simulink model "MMC_phase_hackathon_circuit4_HAAS_20260216"  (R2024b)
settings: Solver=FixedStepDiscrete  StartTime=t_init_sim  StopTime=sim_time  FixedStep=Ts  RelTol=1e-3
values from neighbouring files (symbols this model uses):
  a = 1    [param_phase_circuit4_20260216.m]
  C1low1_active = 1    [script_MMC_phase_circuit4_twist_20260216.m]
  C2low1_active = 1    [script_MMC_phase_circuit4_twist_20260216.m]
  C_bus = 4400e-6    (= 0.0044)    [param_phase_circuit4_20260216.m]
  C_M_extra = C_m-twist_high_side_C    [param_phase_circuit4_20260216.m]
  duty_cycle = 0.95    [script_MMC_phase_circuit4_twist_20260216.m]
  f0 = 50    [param_phase_circuit4_20260216.m]
  feeder_current_lower_rate_limit = -10    [script_MMC_phase_circuit4_twist_20260216.m]    (also in twist_parameters.m = -500)
  feeder_current_tab = [0.328 0.217 0.162 0.132 0.109 0.094 0.083 0.075 0.068 0.062 0.058 0.054 ... (42 elements, 14x3)]    [feeder_current.mat]
  feeder_current_upper_rate_limit = 0.386/(20e-3)    (= 19.3)    [twist_parameters.m]
  is6VExternallySupplied = true    [script_MMC_phase_circuit4_twist_20260216.m]
  isFeederJumperOpen = true    [script_MMC_phase_circuit4_twist_20260216.m]
  L_arm = 30e-3    (= 0.03)    [param_phase_circuit4_20260216.m]
  m = 1    [param_phase_circuit4_20260216.m]
  N = 5    [param_phase_circuit4_20260216.m]
  power_losses = false    [script_MMC_phase_circuit4_twist_20260216.m]
  R = 30    [param_phase_circuit4_20260216.m]
  source_V = 0    [script_MMC_phase_circuit4_twist_20260216.m]
  time_charge = 0.1    [script_MMC_phase_circuit4_twist_20260216.m]
  time_decharge = 1.5    [script_MMC_phase_circuit4_twist_20260216.m]
  Ts = 5e-7    (= 5e-07)    [script_MMC_phase_circuit4_twist_20260216.m]
  twist_data_acquisition_delay = 50e-9    (= 5e-08)    [script_MMC_phase_circuit4_twist_20260216.m]    (also in twist_parameters.m)
  twist_data_sampling_period = 1/twist_freq_data_sampling    (= 5e-05)    [script_MMC_phase_circuit4_twist_20260216.m]    (also in twist_parameters.m)
  twist_dead_time = 200e-9    (= 2e-07)    [twist_parameters.m]
  twist_freq_switching = 200e3    (= 200000)    [twist_parameters.m]
  twist_high_side_adc_R = 1/(1/2e6 + 1/2e6 + 1/(330e3+5.6e3))    (= 251272.836178)    [twist_parameters.m]
  twist_high_side_C = 33e-6*4 + 4.7e-6*12    (= 0.0001884)    [twist_parameters.m]
  twist_high_side_feeder_R = 47e3+4.7e3    (= 51700)    [twist_parameters.m]
  twist_high_side_rC = 0.1    [twist_parameters.m]
  twist_low_side_adc_R = 150e3+470    (= 150470)    [twist_parameters.m]
  twist_low_side_C_ceramic = 3*4.7e-6    (= 1.41e-05)    [twist_parameters.m]
  twist_low_side_C_electrolytic = 47e-6    (= 4.7e-05)    [twist_parameters.m]
  twist_low_side_L = 33e-6    (= 3.3e-05)    [twist_parameters.m]
  twist_low_side_rC = 700e-3    (= 0.7)    [twist_parameters.m]
  twist_low_side_rL = 20e-3    (= 0.02)    [twist_parameters.m]
  twist_R_VCC = (tau_VCC/twist_high_side_C  - twist_high_side_rC)/(1-(tau_VCC/twist_high_side_C - twist_high_side_rC)/R_parallel)    (= 1110.74997822)    [twist_parameters.m]
  VDC = 48    [param_phase_circuit4_20260216.m]
undefined symbols (not defined in the file or in its folder): C_SM, feeder_current, gcbh, sps_rtmsupport, twist_low_side_lC
libraries: spsSeriesRLCBranchLib x135, spsTriangleGeneratorLib x60, spsMosfetLib x60, spsVoltageMeasurementLib x55, spsCurrentMeasurementLib x43, spsControlledCurrentSourceLib x30, spsDiodeLib x22, spsIdealSwitchLib x20, spsControlledVoltageSourceLib x1, spsGroundLib x1, spsMeanLib x1, spspowerguiLib x1
(part 11 of 18)

== system MMC_phase_hackathon_circuit4_HAAS_20260216/ /HB Twist M10/Twist Power Block/HRTimA_1/PWM Generator (2-Level)/Modulator type ==
  Cr : Inport
  Uref : Inport  Port=2
  Full Bridge Bipolar : Subsystem  VariantControl=FullBridgeBipolar
  Full Bridge Unipolar : Subsystem  VariantControl=FullBridgeUnipolar
  One Three Phase Bridge : Subsystem  VariantControl=OneThreePhaseBridge
  P : Outport  VectorParamsAs1DForOutWhenUnconnected=off

== system MMC_phase_hackathon_circuit4_HAAS_20260216/ /HB Twist M10/Twist Power Block/HRTimA_1/PWM Generator (2-Level)/Reference signal ==
  Uref : Inport
  External : Subsystem  VariantControl=External
  Internal : Subsystem  VariantControl=Internal
  Uref_In : Outport  VectorParamsAs1DForOutWhenUnconnected=off

== system MMC_phase_hackathon_circuit4_HAAS_20260216/ /HB Twist M10/Twist Power Block/HRTimA_1/PWM Generator (2-Level)/Sampling ==
  wt : Inport
  Uref : Inport  Port=2
  Sync Asymmetrical : Subsystem  VariantControl=SyncAsymmetrical
  Sync Natural : Subsystem  VariantControl=SyncNatural
  Sync Symmetrical : Subsystem  VariantControl=SyncSymmetrical
  Unsync Asymmetrical : Subsystem  VariantControl=UnsyncAsymmetrical
  Unsync Natural : Subsystem  VariantControl=UnsyncNatural
  Unsync Symmetrical : Subsystem  VariantControl=UnsyncSymmetrical
  Cr : Outport  VectorParamsAs1DForOutWhenUnconnected=off
  Uref* : Outport  Port=2  VectorParamsAs1DForOutWhenUnconnected=off

== system MMC_phase_hackathon_circuit4_HAAS_20260216/ /HB Twist M10/Twist Power Block/HRTimA_2/PWM Generator (2-Level)/Cr_MinMax ==
  MinMax : Inport
  Cr : Inport  Port=2
  Add3 : Sum  Inputs=-+
  Add4 : Sum  Inputs=+++
  Demux : Demux  Outputs=2
  Gain1 : Gain  Gain=0.5
  MUL1 : Product  Inputs=**
  Cr* : Outport  VectorParamsAs1DForOutWhenUnconnected=off
  wires:
  Add3/1 -> Gain1/1
  MinMax/1 -> Demux/1
  Demux/1 -> Add4/1, Add3/1
  Demux/2 -> Add3/2
  Gain1/1 -> Add4/3, MUL1/2
  Cr/1 -> MUL1/1
  Add4/1 -> Cr*/1
  MUL1/1 -> Add4/2

== system MMC_phase_hackathon_circuit4_HAAS_20260216/ /HB Twist M10/Twist Power Block/HRTimA_2/PWM Generator (2-Level)/Modulator type ==
  Cr : Inport
  Uref : Inport  Port=2
  Full Bridge Bipolar : Subsystem  VariantControl=FullBridgeBipolar
  Full Bridge Unipolar : Subsystem  VariantControl=FullBridgeUnipolar
  One Three Phase Bridge : Subsystem  VariantControl=OneThreePhaseBridge
  P : Outport  VectorParamsAs1DForOutWhenUnconnected=off

== system MMC_phase_hackathon_circuit4_HAAS_20260216/ /HB Twist M10/Twist Power Block/HRTimA_2/PWM Generator (2-Level)/Reference signal ==
  Uref : Inport
  External : Subsystem  VariantControl=External
  Internal : Subsystem  VariantControl=Internal
  Uref_In : Outport  VectorParamsAs1DForOutWhenUnconnected=off

== system MMC_phase_hackathon_circuit4_HAAS_20260216/ /HB Twist M10/Twist Power Block/HRTimA_2/PWM Generator (2-Level)/Sampling ==
  wt : Inport
  Uref : Inport  Port=2
  Sync Asymmetrical : Subsystem  VariantControl=SyncAsymmetrical
  Sync Natural : Subsystem  VariantControl=SyncNatural
  Sync Symmetrical : Subsystem  VariantControl=SyncSymmetrical
  Unsync Asymmetrical : Subsystem  VariantControl=UnsyncAsymmetrical
  Unsync Natural : Subsystem  VariantControl=UnsyncNatural
  Unsync Symmetrical : Subsystem  VariantControl=UnsyncSymmetrical
  Cr : Outport  VectorParamsAs1DForOutWhenUnconnected=off
  Uref* : Outport  Port=2  VectorParamsAs1DForOutWhenUnconnected=off

== system MMC_phase_hackathon_circuit4_HAAS_20260216/ /HB Twist M2/Twist Power Block/HRTimA_1/PWM Generator (2-Level)/Cr_MinMax ==
  MinMax : Inport
  Cr : Inport  Port=2
  Add3 : Sum  Inputs=-+
  Add4 : Sum  Inputs=+++
  Demux : Demux  Outputs=2
  Gain1 : Gain  Gain=0.5
  MUL1 : Product  Inputs=**
  Cr* : Outport  VectorParamsAs1DForOutWhenUnconnected=off
  wires:
  Add3/1 -> Gain1/1
  MinMax/1 -> Demux/1
  Demux/1 -> Add4/1, Add3/1
  Demux/2 -> Add3/2
  Gain1/1 -> Add4/3, MUL1/2
  Cr/1 -> MUL1/1
  Add4/1 -> Cr*/1
  MUL1/1 -> Add4/2

== system MMC_phase_hackathon_circuit4_HAAS_20260216/ /HB Twist M2/Twist Power Block/HRTimA_1/PWM Generator (2-Level)/Modulator type ==
  Cr : Inport
  Uref : Inport  Port=2
  Full Bridge Bipolar : Subsystem  VariantControl=FullBridgeBipolar
  Full Bridge Unipolar : Subsystem  VariantControl=FullBridgeUnipolar
  One Three Phase Bridge : Subsystem  VariantControl=OneThreePhaseBridge
  P : Outport  VectorParamsAs1DForOutWhenUnconnected=off

== system MMC_phase_hackathon_circuit4_HAAS_20260216/ /HB Twist M2/Twist Power Block/HRTimA_1/PWM Generator (2-Level)/Reference signal ==
  Uref : Inport
  External : Subsystem  VariantControl=External
  Internal : Subsystem  VariantControl=Internal
  Uref_In : Outport  VectorParamsAs1DForOutWhenUnconnected=off

== system MMC_phase_hackathon_circuit4_HAAS_20260216/ /HB Twist M2/Twist Power Block/HRTimA_1/PWM Generator (2-Level)/Sampling ==
  wt : Inport
  Uref : Inport  Port=2
  Sync Asymmetrical : Subsystem  VariantControl=SyncAsymmetrical
  Sync Natural : Subsystem  VariantControl=SyncNatural
  Sync Symmetrical : Subsystem  VariantControl=SyncSymmetrical
  Unsync Asymmetrical : Subsystem  VariantControl=UnsyncAsymmetrical
  Unsync Natural : Subsystem  VariantControl=UnsyncNatural
  Unsync Symmetrical : Subsystem  VariantControl=UnsyncSymmetrical
  Cr : Outport  VectorParamsAs1DForOutWhenUnconnected=off
  Uref* : Outport  Port=2  VectorParamsAs1DForOutWhenUnconnected=off

== system MMC_phase_hackathon_circuit4_HAAS_20260216/ /HB Twist M2/Twist Power Block/HRTimA_2/PWM Generator (2-Level)/Cr_MinMax ==
  MinMax : Inport
  Cr : Inport  Port=2
  Add3 : Sum  Inputs=-+
  Add4 : Sum  Inputs=+++
  Demux : Demux  Outputs=2
  Gain1 : Gain  Gain=0.5
  MUL1 : Product  Inputs=**
  Cr* : Outport  VectorParamsAs1DForOutWhenUnconnected=off
  wires:
  Add3/1 -> Gain1/1
  MinMax/1 -> Demux/1
  Demux/1 -> Add4/1, Add3/1
  Demux/2 -> Add3/2
  Gain1/1 -> Add4/3, MUL1/2
  Cr/1 -> MUL1/1
  Add4/1 -> Cr*/1
  MUL1/1 -> Add4/2

== system MMC_phase_hackathon_circuit4_HAAS_20260216/ /HB Twist M2/Twist Power Block/HRTimA_2/PWM Generator (2-Level)/Modulator type ==
  Cr : Inport
  Uref : Inport  Port=2
  Full Bridge Bipolar : Subsystem  VariantControl=FullBridgeBipolar
  Full Bridge Unipolar : Subsystem  VariantControl=FullBridgeUnipolar
  One Three Phase Bridge : Subsystem  VariantControl=OneThreePhaseBridge
  P : Outport  VectorParamsAs1DForOutWhenUnconnected=off

== system MMC_phase_hackathon_circuit4_HAAS_20260216/ /HB Twist M2/Twist Power Block/HRTimA_2/PWM Generator (2-Level)/Reference signal ==
  Uref : Inport
  External : Subsystem  VariantControl=External
  Internal : Subsystem  VariantControl=Internal
  Uref_In : Outport  VectorParamsAs1DForOutWhenUnconnected=off

== system MMC_phase_hackathon_circuit4_HAAS_20260216/ /HB Twist M2/Twist Power Block/HRTimA_2/PWM Generator (2-Level)/Sampling ==
  wt : Inport
  Uref : Inport  Port=2
  Sync Asymmetrical : Subsystem  VariantControl=SyncAsymmetrical
  Sync Natural : Subsystem  VariantControl=SyncNatural
  Sync Symmetrical : Subsystem  VariantControl=SyncSymmetrical
  Unsync Asymmetrical : Subsystem  VariantControl=UnsyncAsymmetrical
  Unsync Natural : Subsystem  VariantControl=UnsyncNatural
  Unsync Symmetrical : Subsystem  VariantControl=UnsyncSymmetrical
  Cr : Outport  VectorParamsAs1DForOutWhenUnconnected=off
  Uref* : Outport  Port=2  VectorParamsAs1DForOutWhenUnconnected=off

== system MMC_phase_hackathon_circuit4_HAAS_20260216/ /HB Twist M3/Twist Power Block/HRTimA_1/PWM Generator (2-Level)/Cr_MinMax ==
  MinMax : Inport
  Cr : Inport  Port=2
  Add3 : Sum  Inputs=-+
  Add4 : Sum  Inputs=+++
  Demux : Demux  Outputs=2
  Gain1 : Gain  Gain=0.5
  MUL1 : Product  Inputs=**
  Cr* : Outport  VectorParamsAs1DForOutWhenUnconnected=off
  wires:
  Add3/1 -> Gain1/1
  MinMax/1 -> Demux/1
  Demux/1 -> Add4/1, Add3/1
  Demux/2 -> Add3/2
  Gain1/1 -> Add4/3, MUL1/2
  Cr/1 -> MUL1/1
  Add4/1 -> Cr*/1
  MUL1/1 -> Add4/2

== system MMC_phase_hackathon_circuit4_HAAS_20260216/ /HB Twist M3/Twist Power Block/HRTimA_1/PWM Generator (2-Level)/Modulator type ==
  Cr : Inport
  Uref : Inport  Port=2
  Full Bridge Bipolar : Subsystem  VariantControl=FullBridgeBipolar
  Full Bridge Unipolar : Subsystem  VariantControl=FullBridgeUnipolar
  One Three Phase Bridge : Subsystem  VariantControl=OneThreePhaseBridge
  P : Outport  VectorParamsAs1DForOutWhenUnconnected=off

== system MMC_phase_hackathon_circuit4_HAAS_20260216/ /HB Twist M3/Twist Power Block/HRTimA_1/PWM Generator (2-Level)/Reference signal ==
  Uref : Inport
  External : Subsystem  VariantControl=External
  Internal : Subsystem  VariantControl=Internal
  Uref_In : Outport  VectorParamsAs1DForOutWhenUnconnected=off

== system MMC_phase_hackathon_circuit4_HAAS_20260216/ /HB Twist M3/Twist Power Block/HRTimA_1/PWM Generator (2-Level)/Sampling ==
  wt : Inport
  Uref : Inport  Port=2
  Sync Asymmetrical : Subsystem  VariantControl=SyncAsymmetrical
  Sync Natural : Subsystem  VariantControl=SyncNatural
  Sync Symmetrical : Subsystem  VariantControl=SyncSymmetrical
  Unsync Asymmetrical : Subsystem  VariantControl=UnsyncAsymmetrical
  Unsync Natural : Subsystem  VariantControl=UnsyncNatural
  Unsync Symmetrical : Subsystem  VariantControl=UnsyncSymmetrical
  Cr : Outport  VectorParamsAs1DForOutWhenUnconnected=off
  Uref* : Outport  Port=2  VectorParamsAs1DForOutWhenUnconnected=off

== system MMC_phase_hackathon_circuit4_HAAS_20260216/ /HB Twist M3/Twist Power Block/HRTimA_2/PWM Generator (2-Level)/Cr_MinMax ==
  MinMax : Inport
  Cr : Inport  Port=2
  Add3 : Sum  Inputs=-+
  Add4 : Sum  Inputs=+++
  Demux : Demux  Outputs=2
  Gain1 : Gain  Gain=0.5
  MUL1 : Product  Inputs=**
  Cr* : Outport  VectorParamsAs1DForOutWhenUnconnected=off
  wires:
  Add3/1 -> Gain1/1
  MinMax/1 -> Demux/1
  Demux/1 -> Add4/1, Add3/1
  Demux/2 -> Add3/2
  Gain1/1 -> Add4/3, MUL1/2
  Cr/1 -> MUL1/1
  Add4/1 -> Cr*/1
  MUL1/1 -> Add4/2

== system MMC_phase_hackathon_circuit4_HAAS_20260216/ /HB Twist M3/Twist Power Block/HRTimA_2/PWM Generator (2-Level)/Modulator type ==
  Cr : Inport
  Uref : Inport  Port=2
  Full Bridge Bipolar : Subsystem  VariantControl=FullBridgeBipolar
  Full Bridge Unipolar : Subsystem  VariantControl=FullBridgeUnipolar
  One Three Phase Bridge : Subsystem  VariantControl=OneThreePhaseBridge
  P : Outport  VectorParamsAs1DForOutWhenUnconnected=off

== system MMC_phase_hackathon_circuit4_HAAS_20260216/ /HB Twist M3/Twist Power Block/HRTimA_2/PWM Generator (2-Level)/Reference signal ==
  Uref : Inport
  External : Subsystem  VariantControl=External
  Internal : Subsystem  VariantControl=Internal
  Uref_In : Outport  VectorParamsAs1DForOutWhenUnconnected=off

== system MMC_phase_hackathon_circuit4_HAAS_20260216/ /HB Twist M3/Twist Power Block/HRTimA_2/PWM Generator (2-Level)/Sampling ==
  wt : Inport
  Uref : Inport  Port=2
  Sync Asymmetrical : Subsystem  VariantControl=SyncAsymmetrical
  Sync Natural : Subsystem  VariantControl=SyncNatural
  Sync Symmetrical : Subsystem  VariantControl=SyncSymmetrical
  Unsync Asymmetrical : Subsystem  VariantControl=UnsyncAsymmetrical
  Unsync Natural : Subsystem  VariantControl=UnsyncNatural
  Unsync Symmetrical : Subsystem  VariantControl=UnsyncSymmetrical
  Cr : Outport  VectorParamsAs1DForOutWhenUnconnected=off
  Uref* : Outport  Port=2  VectorParamsAs1DForOutWhenUnconnected=off

== system MMC_phase_hackathon_circuit4_HAAS_20260216/ /HB Twist M4/Twist Power Block/HRTimA_1/PWM Generator (2-Level)/Cr_MinMax ==
  MinMax : Inport
  Cr : Inport  Port=2
  Add3 : Sum  Inputs=-+
  Add4 : Sum  Inputs=+++
  Demux : Demux  Outputs=2
  Gain1 : Gain  Gain=0.5
  MUL1 : Product  Inputs=**
  Cr* : Outport  VectorParamsAs1DForOutWhenUnconnected=off
  wires:
  Add3/1 -> Gain1/1
  MinMax/1 -> Demux/1
  Demux/1 -> Add4/1, Add3/1
  Demux/2 -> Add3/2
  Gain1/1 -> Add4/3, MUL1/2
  Cr/1 -> MUL1/1
  Add4/1 -> Cr*/1
  MUL1/1 -> Add4/2

== system MMC_phase_hackathon_circuit4_HAAS_20260216/ /HB Twist M4/Twist Power Block/HRTimA_1/PWM Generator (2-Level)/Modulator type ==
  Cr : Inport
  Uref : Inport  Port=2
  Full Bridge Bipolar : Subsystem  VariantControl=FullBridgeBipolar
  Full Bridge Unipolar : Subsystem  VariantControl=FullBridgeUnipolar
  One Three Phase Bridge : Subsystem  VariantControl=OneThreePhaseBridge
  P : Outport  VectorParamsAs1DForOutWhenUnconnected=off

== system MMC_phase_hackathon_circuit4_HAAS_20260216/ /HB Twist M4/Twist Power Block/HRTimA_1/PWM Generator (2-Level)/Reference signal ==
  Uref : Inport
  External : Subsystem  VariantControl=External
  Internal : Subsystem  VariantControl=Internal
  Uref_In : Outport  VectorParamsAs1DForOutWhenUnconnected=off

== system MMC_phase_hackathon_circuit4_HAAS_20260216/ /HB Twist M4/Twist Power Block/HRTimA_1/PWM Generator (2-Level)/Sampling ==
  wt : Inport
  Uref : Inport  Port=2
  Sync Asymmetrical : Subsystem  VariantControl=SyncAsymmetrical
  Sync Natural : Subsystem  VariantControl=SyncNatural
  Sync Symmetrical : Subsystem  VariantControl=SyncSymmetrical
  Unsync Asymmetrical : Subsystem  VariantControl=UnsyncAsymmetrical
  Unsync Natural : Subsystem  VariantControl=UnsyncNatural
  Unsync Symmetrical : Subsystem  VariantControl=UnsyncSymmetrical
  Cr : Outport  VectorParamsAs1DForOutWhenUnconnected=off
  Uref* : Outport  Port=2  VectorParamsAs1DForOutWhenUnconnected=off

== system MMC_phase_hackathon_circuit4_HAAS_20260216/ /HB Twist M4/Twist Power Block/HRTimA_2/PWM Generator (2-Level)/Cr_MinMax ==
  MinMax : Inport
  Cr : Inport  Port=2
  Add3 : Sum  Inputs=-+
  Add4 : Sum  Inputs=+++
  Demux : Demux  Outputs=2
  Gain1 : Gain  Gain=0.5
  MUL1 : Product  Inputs=**
  Cr* : Outport  VectorParamsAs1DForOutWhenUnconnected=off
  wires:
  Add3/1 -> Gain1/1
  MinMax/1 -> Demux/1
  Demux/1 -> Add4/1, Add3/1
  Demux/2 -> Add3/2
  Gain1/1 -> Add4/3, MUL1/2
  Cr/1 -> MUL1/1
  Add4/1 -> Cr*/1
  MUL1/1 -> Add4/2

== system MMC_phase_hackathon_circuit4_HAAS_20260216/ /HB Twist M4/Twist Power Block/HRTimA_2/PWM Generator (2-Level)/Modulator type ==
  Cr : Inport
  Uref : Inport  Port=2
  Full Bridge Bipolar : Subsystem  VariantControl=FullBridgeBipolar
  Full Bridge Unipolar : Subsystem  VariantControl=FullBridgeUnipolar
  One Three Phase Bridge : Subsystem  VariantControl=OneThreePhaseBridge
  P : Outport  VectorParamsAs1DForOutWhenUnconnected=off

== system MMC_phase_hackathon_circuit4_HAAS_20260216/ /HB Twist M4/Twist Power Block/HRTimA_2/PWM Generator (2-Level)/Reference signal ==
  Uref : Inport
  External : Subsystem  VariantControl=External
  Internal : Subsystem  VariantControl=Internal
  Uref_In : Outport  VectorParamsAs1DForOutWhenUnconnected=off

== system MMC_phase_hackathon_circuit4_HAAS_20260216/ /HB Twist M4/Twist Power Block/HRTimA_2/PWM Generator (2-Level)/Sampling ==
  wt : Inport
  Uref : Inport  Port=2
  Sync Asymmetrical : Subsystem  VariantControl=SyncAsymmetrical
  Sync Natural : Subsystem  VariantControl=SyncNatural
  Sync Symmetrical : Subsystem  VariantControl=SyncSymmetrical
  Unsync Asymmetrical : Subsystem  VariantControl=UnsyncAsymmetrical
  Unsync Natural : Subsystem  VariantControl=UnsyncNatural
  Unsync Symmetrical : Subsystem  VariantControl=UnsyncSymmetrical
  Cr : Outport  VectorParamsAs1DForOutWhenUnconnected=off
  Uref* : Outport  Port=2  VectorParamsAs1DForOutWhenUnconnected=off

== system MMC_phase_hackathon_circuit4_HAAS_20260216/ /HB Twist M5/Twist Power Block/HRTimA_1/PWM Generator (2-Level)/Cr_MinMax ==
  MinMax : Inport
  Cr : Inport  Port=2
  Add3 : Sum  Inputs=-+
  Add4 : Sum  Inputs=+++
  Demux : Demux  Outputs=2
  Gain1 : Gain  Gain=0.5
  MUL1 : Product  Inputs=**
  Cr* : Outport  VectorParamsAs1DForOutWhenUnconnected=off
  wires:
  Add3/1 -> Gain1/1
  MinMax/1 -> Demux/1
  Demux/1 -> Add4/1, Add3/1
  Demux/2 -> Add3/2
  Gain1/1 -> Add4/3, MUL1/2
  Cr/1 -> MUL1/1
  Add4/1 -> Cr*/1
  MUL1/1 -> Add4/2

== system MMC_phase_hackathon_circuit4_HAAS_20260216/ /HB Twist M5/Twist Power Block/HRTimA_1/PWM Generator (2-Level)/Modulator type ==
  Cr : Inport
  Uref : Inport  Port=2
  Full Bridge Bipolar : Subsystem  VariantControl=FullBridgeBipolar
  Full Bridge Unipolar : Subsystem  VariantControl=FullBridgeUnipolar
  One Three Phase Bridge : Subsystem  VariantControl=OneThreePhaseBridge
  P : Outport  VectorParamsAs1DForOutWhenUnconnected=off

== system MMC_phase_hackathon_circuit4_HAAS_20260216/ /HB Twist M5/Twist Power Block/HRTimA_1/PWM Generator (2-Level)/Reference signal ==
  Uref : Inport
  External : Subsystem  VariantControl=External
  Internal : Subsystem  VariantControl=Internal
  Uref_In : Outport  VectorParamsAs1DForOutWhenUnconnected=off

== system MMC_phase_hackathon_circuit4_HAAS_20260216/ /HB Twist M5/Twist Power Block/HRTimA_1/PWM Generator (2-Level)/Sampling ==
  wt : Inport
  Uref : Inport  Port=2
  Sync Asymmetrical : Subsystem  VariantControl=SyncAsymmetrical
  Sync Natural : Subsystem  VariantControl=SyncNatural
  Sync Symmetrical : Subsystem  VariantControl=SyncSymmetrical
  Unsync Asymmetrical : Subsystem  VariantControl=UnsyncAsymmetrical
  Unsync Natural : Subsystem  VariantControl=UnsyncNatural
  Unsync Symmetrical : Subsystem  VariantControl=UnsyncSymmetrical
  Cr : Outport  VectorParamsAs1DForOutWhenUnconnected=off
  Uref* : Outport  Port=2  VectorParamsAs1DForOutWhenUnconnected=off

== system MMC_phase_hackathon_circuit4_HAAS_20260216/ /HB Twist M5/Twist Power Block/HRTimA_2/PWM Generator (2-Level)/Cr_MinMax ==
  MinMax : Inport
  Cr : Inport  Port=2
  Add3 : Sum  Inputs=-+
  Add4 : Sum  Inputs=+++
  Demux : Demux  Outputs=2
  Gain1 : Gain  Gain=0.5
  MUL1 : Product  Inputs=**
  Cr* : Outport  VectorParamsAs1DForOutWhenUnconnected=off
  wires:
  Add3/1 -> Gain1/1
  MinMax/1 -> Demux/1
  Demux/1 -> Add4/1, Add3/1
  Demux/2 -> Add3/2
  Gain1/1 -> Add4/3, MUL1/2
  Cr/1 -> MUL1/1
  Add4/1 -> Cr*/1
  MUL1/1 -> Add4/2

== system MMC_phase_hackathon_circuit4_HAAS_20260216/ /HB Twist M5/Twist Power Block/HRTimA_2/PWM Generator (2-Level)/Modulator type ==
  Cr : Inport
  Uref : Inport  Port=2
  Full Bridge Bipolar : Subsystem  VariantControl=FullBridgeBipolar
  Full Bridge Unipolar : Subsystem  VariantControl=FullBridgeUnipolar
  One Three Phase Bridge : Subsystem  VariantControl=OneThreePhaseBridge
  P : Outport  VectorParamsAs1DForOutWhenUnconnected=off

== system MMC_phase_hackathon_circuit4_HAAS_20260216/ /HB Twist M5/Twist Power Block/HRTimA_2/PWM Generator (2-Level)/Reference signal ==
  Uref : Inport
  External : Subsystem  VariantControl=External
  Internal : Subsystem  VariantControl=Internal
  Uref_In : Outport  VectorParamsAs1DForOutWhenUnconnected=off

== system MMC_phase_hackathon_circuit4_HAAS_20260216/ /HB Twist M5/Twist Power Block/HRTimA_2/PWM Generator (2-Level)/Sampling ==
  wt : Inport
  Uref : Inport  Port=2
  Sync Asymmetrical : Subsystem  VariantControl=SyncAsymmetrical
  Sync Natural : Subsystem  VariantControl=SyncNatural
  Sync Symmetrical : Subsystem  VariantControl=SyncSymmetrical
  Unsync Asymmetrical : Subsystem  VariantControl=UnsyncAsymmetrical
  Unsync Natural : Subsystem  VariantControl=UnsyncNatural
  Unsync Symmetrical : Subsystem  VariantControl=UnsyncSymmetrical
  Cr : Outport  VectorParamsAs1DForOutWhenUnconnected=off
  Uref* : Outport  Port=2  VectorParamsAs1DForOutWhenUnconnected=off

== system MMC_phase_hackathon_circuit4_HAAS_20260216/ /HB Twist M6/Twist Power Block/HRTimA_1/PWM Generator (2-Level)/Cr_MinMax ==
  MinMax : Inport
  Cr : Inport  Port=2
  Add3 : Sum  Inputs=-+
  Add4 : Sum  Inputs=+++
  Demux : Demux  Outputs=2
  Gain1 : Gain  Gain=0.5
  MUL1 : Product  Inputs=**
  Cr* : Outport  VectorParamsAs1DForOutWhenUnconnected=off
  wires:
  Add3/1 -> Gain1/1
  MinMax/1 -> Demux/1
  Demux/1 -> Add4/1, Add3/1
  Demux/2 -> Add3/2
  Gain1/1 -> Add4/3, MUL1/2
  Cr/1 -> MUL1/1
  Add4/1 -> Cr*/1
  MUL1/1 -> Add4/2

== system MMC_phase_hackathon_circuit4_HAAS_20260216/ /HB Twist M6/Twist Power Block/HRTimA_1/PWM Generator (2-Level)/Modulator type ==
  Cr : Inport
  Uref : Inport  Port=2
  Full Bridge Bipolar : Subsystem  VariantControl=FullBridgeBipolar
  Full Bridge Unipolar : Subsystem  VariantControl=FullBridgeUnipolar
  One Three Phase Bridge : Subsystem  VariantControl=OneThreePhaseBridge
  P : Outport  VectorParamsAs1DForOutWhenUnconnected=off

== system MMC_phase_hackathon_circuit4_HAAS_20260216/ /HB Twist M6/Twist Power Block/HRTimA_1/PWM Generator (2-Level)/Reference signal ==
  Uref : Inport
  External : Subsystem  VariantControl=External
  Internal : Subsystem  VariantControl=Internal
  Uref_In : Outport  VectorParamsAs1DForOutWhenUnconnected=off

== system MMC_phase_hackathon_circuit4_HAAS_20260216/ /HB Twist M6/Twist Power Block/HRTimA_1/PWM Generator (2-Level)/Sampling ==
  wt : Inport
  Uref : Inport  Port=2
  Sync Asymmetrical : Subsystem  VariantControl=SyncAsymmetrical
  Sync Natural : Subsystem  VariantControl=SyncNatural
  Sync Symmetrical : Subsystem  VariantControl=SyncSymmetrical
  Unsync Asymmetrical : Subsystem  VariantControl=UnsyncAsymmetrical
  Unsync Natural : Subsystem  VariantControl=UnsyncNatural
  Unsync Symmetrical : Subsystem  VariantControl=UnsyncSymmetrical
  Cr : Outport  VectorParamsAs1DForOutWhenUnconnected=off
  Uref* : Outport  Port=2  VectorParamsAs1DForOutWhenUnconnected=off

== system MMC_phase_hackathon_circuit4_HAAS_20260216/ /HB Twist M6/Twist Power Block/HRTimA_2/PWM Generator (2-Level)/Cr_MinMax ==
  MinMax : Inport
  Cr : Inport  Port=2
  Add3 : Sum  Inputs=-+
  Add4 : Sum  Inputs=+++
  Demux : Demux  Outputs=2
  Gain1 : Gain  Gain=0.5
  MUL1 : Product  Inputs=**
  Cr* : Outport  VectorParamsAs1DForOutWhenUnconnected=off
  wires:
  Add3/1 -> Gain1/1
  MinMax/1 -> Demux/1
  Demux/1 -> Add4/1, Add3/1
  Demux/2 -> Add3/2
  Gain1/1 -> Add4/3, MUL1/2
  Cr/1 -> MUL1/1
  Add4/1 -> Cr*/1
  MUL1/1 -> Add4/2

== system MMC_phase_hackathon_circuit4_HAAS_20260216/ /HB Twist M6/Twist Power Block/HRTimA_2/PWM Generator (2-Level)/Modulator type ==
  Cr : Inport
  Uref : Inport  Port=2
  Full Bridge Bipolar : Subsystem  VariantControl=FullBridgeBipolar
  Full Bridge Unipolar : Subsystem  VariantControl=FullBridgeUnipolar
  One Three Phase Bridge : Subsystem  VariantControl=OneThreePhaseBridge
  P : Outport  VectorParamsAs1DForOutWhenUnconnected=off

== system MMC_phase_hackathon_circuit4_HAAS_20260216/ /HB Twist M6/Twist Power Block/HRTimA_2/PWM Generator (2-Level)/Reference signal ==
  Uref : Inport
  External : Subsystem  VariantControl=External
  Internal : Subsystem  VariantControl=Internal
  Uref_In : Outport  VectorParamsAs1DForOutWhenUnconnected=off

== system MMC_phase_hackathon_circuit4_HAAS_20260216/ /HB Twist M6/Twist Power Block/HRTimA_2/PWM Generator (2-Level)/Sampling ==
  wt : Inport
  Uref : Inport  Port=2
  Sync Asymmetrical : Subsystem  VariantControl=SyncAsymmetrical
  Sync Natural : Subsystem  VariantControl=SyncNatural
  Sync Symmetrical : Subsystem  VariantControl=SyncSymmetrical
  Unsync Asymmetrical : Subsystem  VariantControl=UnsyncAsymmetrical
  Unsync Natural : Subsystem  VariantControl=UnsyncNatural
  Unsync Symmetrical : Subsystem  VariantControl=UnsyncSymmetrical
  Cr : Outport  VectorParamsAs1DForOutWhenUnconnected=off
  Uref* : Outport  Port=2  VectorParamsAs1DForOutWhenUnconnected=off

== system MMC_phase_hackathon_circuit4_HAAS_20260216/ /HB Twist M7/Twist Power Block/HRTimA_1/PWM Generator (2-Level)/Cr_MinMax ==
  MinMax : Inport
  Cr : Inport  Port=2
  Add3 : Sum  Inputs=-+
  Add4 : Sum  Inputs=+++
  Demux : Demux  Outputs=2
  Gain1 : Gain  Gain=0.5
  MUL1 : Product  Inputs=**
  Cr* : Outport  VectorParamsAs1DForOutWhenUnconnected=off
  wires:
  Add3/1 -> Gain1/1
  MinMax/1 -> Demux/1
  Demux/1 -> Add4/1, Add3/1
  Demux/2 -> Add3/2
  Gain1/1 -> Add4/3, MUL1/2
  Cr/1 -> MUL1/1
  Add4/1 -> Cr*/1
  MUL1/1 -> Add4/2

== system MMC_phase_hackathon_circuit4_HAAS_20260216/ /HB Twist M7/Twist Power Block/HRTimA_1/PWM Generator (2-Level)/Modulator type ==
  Cr : Inport
  Uref : Inport  Port=2
  Full Bridge Bipolar : Subsystem  VariantControl=FullBridgeBipolar
  Full Bridge Unipolar : Subsystem  VariantControl=FullBridgeUnipolar
  One Three Phase Bridge : Subsystem  VariantControl=OneThreePhaseBridge
  P : Outport  VectorParamsAs1DForOutWhenUnconnected=off

== system MMC_phase_hackathon_circuit4_HAAS_20260216/ /HB Twist M7/Twist Power Block/HRTimA_1/PWM Generator (2-Level)/Reference signal ==
  Uref : Inport
  External : Subsystem  VariantControl=External
  Internal : Subsystem  VariantControl=Internal
  Uref_In : Outport  VectorParamsAs1DForOutWhenUnconnected=off

== system MMC_phase_hackathon_circuit4_HAAS_20260216/ /HB Twist M7/Twist Power Block/HRTimA_1/PWM Generator (2-Level)/Sampling ==
  wt : Inport
  Uref : Inport  Port=2
  Sync Asymmetrical : Subsystem  VariantControl=SyncAsymmetrical
  Sync Natural : Subsystem  VariantControl=SyncNatural
  Sync Symmetrical : Subsystem  VariantControl=SyncSymmetrical
  Unsync Asymmetrical : Subsystem  VariantControl=UnsyncAsymmetrical
  Unsync Natural : Subsystem  VariantControl=UnsyncNatural
  Unsync Symmetrical : Subsystem  VariantControl=UnsyncSymmetrical
  Cr : Outport  VectorParamsAs1DForOutWhenUnconnected=off
  Uref* : Outport  Port=2  VectorParamsAs1DForOutWhenUnconnected=off

== system MMC_phase_hackathon_circuit4_HAAS_20260216/ /HB Twist M7/Twist Power Block/HRTimA_2/PWM Generator (2-Level)/Cr_MinMax ==
  MinMax : Inport
  Cr : Inport  Port=2
  Add3 : Sum  Inputs=-+
  Add4 : Sum  Inputs=+++
  Demux : Demux  Outputs=2
  Gain1 : Gain  Gain=0.5
  MUL1 : Product  Inputs=**
  Cr* : Outport  VectorParamsAs1DForOutWhenUnconnected=off
  wires:
  Add3/1 -> Gain1/1
  MinMax/1 -> Demux/1
  Demux/1 -> Add4/1, Add3/1
  Demux/2 -> Add3/2
  Gain1/1 -> Add4/3, MUL1/2
  Cr/1 -> MUL1/1
  Add4/1 -> Cr*/1
  MUL1/1 -> Add4/2

== system MMC_phase_hackathon_circuit4_HAAS_20260216/ /HB Twist M7/Twist Power Block/HRTimA_2/PWM Generator (2-Level)/Modulator type ==
  Cr : Inport
  Uref : Inport  Port=2
  Full Bridge Bipolar : Subsystem  VariantControl=FullBridgeBipolar
  Full Bridge Unipolar : Subsystem  VariantControl=FullBridgeUnipolar
  One Three Phase Bridge : Subsystem  VariantControl=OneThreePhaseBridge
  P : Outport  VectorParamsAs1DForOutWhenUnconnected=off

== system MMC_phase_hackathon_circuit4_HAAS_20260216/ /HB Twist M7/Twist Power Block/HRTimA_2/PWM Generator (2-Level)/Reference signal ==
  Uref : Inport
  External : Subsystem  VariantControl=External
  Internal : Subsystem  VariantControl=Internal
  Uref_In : Outport  VectorParamsAs1DForOutWhenUnconnected=off

== system MMC_phase_hackathon_circuit4_HAAS_20260216/ /HB Twist M7/Twist Power Block/HRTimA_2/PWM Generator (2-Level)/Sampling ==
  wt : Inport
  Uref : Inport  Port=2
  Sync Asymmetrical : Subsystem  VariantControl=SyncAsymmetrical
  Sync Natural : Subsystem  VariantControl=SyncNatural
  Sync Symmetrical : Subsystem  VariantControl=SyncSymmetrical
  Unsync Asymmetrical : Subsystem  VariantControl=UnsyncAsymmetrical
  Unsync Natural : Subsystem  VariantControl=UnsyncNatural
  Unsync Symmetrical : Subsystem  VariantControl=UnsyncSymmetrical
  Cr : Outport  VectorParamsAs1DForOutWhenUnconnected=off
  Uref* : Outport  Port=2  VectorParamsAs1DForOutWhenUnconnected=off

== system MMC_phase_hackathon_circuit4_HAAS_20260216/ /HB Twist M8/Twist Power Block/HRTimA_1/PWM Generator (2-Level)/Cr_MinMax ==
  MinMax : Inport
  Cr : Inport  Port=2
  Add3 : Sum  Inputs=-+
  Add4 : Sum  Inputs=+++
  Demux : Demux  Outputs=2
  Gain1 : Gain  Gain=0.5
  MUL1 : Product  Inputs=**
  Cr* : Outport  VectorParamsAs1DForOutWhenUnconnected=off
  wires:
  Add3/1 -> Gain1/1
  MinMax/1 -> Demux/1
  Demux/1 -> Add4/1, Add3/1
  Demux/2 -> Add3/2
  Gain1/1 -> Add4/3, MUL1/2
  Cr/1 -> MUL1/1
  Add4/1 -> Cr*/1
  MUL1/1 -> Add4/2

== system MMC_phase_hackathon_circuit4_HAAS_20260216/ /HB Twist M8/Twist Power Block/HRTimA_1/PWM Generator (2-Level)/Modulator type ==
  Cr : Inport
  Uref : Inport  Port=2
  Full Bridge Bipolar : Subsystem  VariantControl=FullBridgeBipolar
  Full Bridge Unipolar : Subsystem  VariantControl=FullBridgeUnipolar
  One Three Phase Bridge : Subsystem  VariantControl=OneThreePhaseBridge
  P : Outport  VectorParamsAs1DForOutWhenUnconnected=off

== system MMC_phase_hackathon_circuit4_HAAS_20260216/ /HB Twist M8/Twist Power Block/HRTimA_1/PWM Generator (2-Level)/Reference signal ==
  Uref : Inport
  External : Subsystem  VariantControl=External
  Internal : Subsystem  VariantControl=Internal
  Uref_In : Outport  VectorParamsAs1DForOutWhenUnconnected=off

== system MMC_phase_hackathon_circuit4_HAAS_20260216/ /HB Twist M8/Twist Power Block/HRTimA_1/PWM Generator (2-Level)/Sampling ==
  wt : Inport
  Uref : Inport  Port=2
  Sync Asymmetrical : Subsystem  VariantControl=SyncAsymmetrical
  Sync Natural : Subsystem  VariantControl=SyncNatural
  Sync Symmetrical : Subsystem  VariantControl=SyncSymmetrical
  Unsync Asymmetrical : Subsystem  VariantControl=UnsyncAsymmetrical
  Unsync Natural : Subsystem  VariantControl=UnsyncNatural
  Unsync Symmetrical : Subsystem  VariantControl=UnsyncSymmetrical
  Cr : Outport  VectorParamsAs1DForOutWhenUnconnected=off
  Uref* : Outport  Port=2  VectorParamsAs1DForOutWhenUnconnected=off

== system MMC_phase_hackathon_circuit4_HAAS_20260216/ /HB Twist M8/Twist Power Block/HRTimA_2/PWM Generator (2-Level)/Cr_MinMax ==
  MinMax : Inport
  Cr : Inport  Port=2
  Add3 : Sum  Inputs=-+
  Add4 : Sum  Inputs=+++
  Demux : Demux  Outputs=2
  Gain1 : Gain  Gain=0.5
  MUL1 : Product  Inputs=**
  Cr* : Outport  VectorParamsAs1DForOutWhenUnconnected=off
  wires:
  Add3/1 -> Gain1/1
  MinMax/1 -> Demux/1
  Demux/1 -> Add4/1, Add3/1
  Demux/2 -> Add3/2
  Gain1/1 -> Add4/3, MUL1/2
  Cr/1 -> MUL1/1
  Add4/1 -> Cr*/1
  MUL1/1 -> Add4/2

== system MMC_phase_hackathon_circuit4_HAAS_20260216/ /HB Twist M8/Twist Power Block/HRTimA_2/PWM Generator (2-Level)/Modulator type ==
  Cr : Inport
  Uref : Inport  Port=2
  Full Bridge Bipolar : Subsystem  VariantControl=FullBridgeBipolar
  Full Bridge Unipolar : Subsystem  VariantControl=FullBridgeUnipolar
  One Three Phase Bridge : Subsystem  VariantControl=OneThreePhaseBridge
  P : Outport  VectorParamsAs1DForOutWhenUnconnected=off

== system MMC_phase_hackathon_circuit4_HAAS_20260216/ /HB Twist M8/Twist Power Block/HRTimA_2/PWM Generator (2-Level)/Reference signal ==
  Uref : Inport
  External : Subsystem  VariantControl=External
  Internal : Subsystem  VariantControl=Internal
  Uref_In : Outport  VectorParamsAs1DForOutWhenUnconnected=off

== system MMC_phase_hackathon_circuit4_HAAS_20260216/ /HB Twist M8/Twist Power Block/HRTimA_2/PWM Generator (2-Level)/Sampling ==
  wt : Inport
  Uref : Inport  Port=2
  Sync Asymmetrical : Subsystem  VariantControl=SyncAsymmetrical
  Sync Natural : Subsystem  VariantControl=SyncNatural
  Sync Symmetrical : Subsystem  VariantControl=SyncSymmetrical
  Unsync Asymmetrical : Subsystem  VariantControl=UnsyncAsymmetrical
  Unsync Natural : Subsystem  VariantControl=UnsyncNatural
  Unsync Symmetrical : Subsystem  VariantControl=UnsyncSymmetrical
  Cr : Outport  VectorParamsAs1DForOutWhenUnconnected=off
  Uref* : Outport  Port=2  VectorParamsAs1DForOutWhenUnconnected=off

== system MMC_phase_hackathon_circuit4_HAAS_20260216/ /HB Twist M9/Twist Power Block/HRTimA_1/PWM Generator (2-Level)/Cr_MinMax ==
  MinMax : Inport
  Cr : Inport  Port=2
  Add3 : Sum  Inputs=-+
  Add4 : Sum  Inputs=+++
  Demux : Demux  Outputs=2
  Gain1 : Gain  Gain=0.5
  MUL1 : Product  Inputs=**
  Cr* : Outport  VectorParamsAs1DForOutWhenUnconnected=off
  wires:
  Add3/1 -> Gain1/1
  MinMax/1 -> Demux/1
  Demux/1 -> Add4/1, Add3/1
  Demux/2 -> Add3/2
  Gain1/1 -> Add4/3, MUL1/2
  Cr/1 -> MUL1/1
  Add4/1 -> Cr*/1
  MUL1/1 -> Add4/2

== system MMC_phase_hackathon_circuit4_HAAS_20260216/ /HB Twist M9/Twist Power Block/HRTimA_1/PWM Generator (2-Level)/Modulator type ==
  Cr : Inport
  Uref : Inport  Port=2
  Full Bridge Bipolar : Subsystem  VariantControl=FullBridgeBipolar
  Full Bridge Unipolar : Subsystem  VariantControl=FullBridgeUnipolar
  One Three Phase Bridge : Subsystem  VariantControl=OneThreePhaseBridge
  P : Outport  VectorParamsAs1DForOutWhenUnconnected=off

== system MMC_phase_hackathon_circuit4_HAAS_20260216/ /HB Twist M9/Twist Power Block/HRTimA_1/PWM Generator (2-Level)/Reference signal ==
  Uref : Inport
  External : Subsystem  VariantControl=External
  Internal : Subsystem  VariantControl=Internal
  Uref_In : Outport  VectorParamsAs1DForOutWhenUnconnected=off

== system MMC_phase_hackathon_circuit4_HAAS_20260216/ /HB Twist M9/Twist Power Block/HRTimA_1/PWM Generator (2-Level)/Sampling ==
  wt : Inport
  Uref : Inport  Port=2
  Sync Asymmetrical : Subsystem  VariantControl=SyncAsymmetrical
  Sync Natural : Subsystem  VariantControl=SyncNatural
  Sync Symmetrical : Subsystem  VariantControl=SyncSymmetrical
  Unsync Asymmetrical : Subsystem  VariantControl=UnsyncAsymmetrical
  Unsync Natural : Subsystem  VariantControl=UnsyncNatural
  Unsync Symmetrical : Subsystem  VariantControl=UnsyncSymmetrical
  Cr : Outport  VectorParamsAs1DForOutWhenUnconnected=off
  Uref* : Outport  Port=2  VectorParamsAs1DForOutWhenUnconnected=off

== system MMC_phase_hackathon_circuit4_HAAS_20260216/ /HB Twist M9/Twist Power Block/HRTimA_2/PWM Generator (2-Level)/Cr_MinMax ==
  MinMax : Inport
  Cr : Inport  Port=2
  Add3 : Sum  Inputs=-+
  Add4 : Sum  Inputs=+++
  Demux : Demux  Outputs=2
  Gain1 : Gain  Gain=0.5
  MUL1 : Product  Inputs=**
  Cr* : Outport  VectorParamsAs1DForOutWhenUnconnected=off
  wires:
  Add3/1 -> Gain1/1
  MinMax/1 -> Demux/1
  Demux/1 -> Add4/1, Add3/1
  Demux/2 -> Add3/2
  Gain1/1 -> Add4/3, MUL1/2
  Cr/1 -> MUL1/1
  Add4/1 -> Cr*/1
  MUL1/1 -> Add4/2

== system MMC_phase_hackathon_circuit4_HAAS_20260216/ /HB Twist M9/Twist Power Block/HRTimA_2/PWM Generator (2-Level)/Modulator type ==
  Cr : Inport
  Uref : Inport  Port=2
  Full Bridge Bipolar : Subsystem  VariantControl=FullBridgeBipolar
  Full Bridge Unipolar : Subsystem  VariantControl=FullBridgeUnipolar
  One Three Phase Bridge : Subsystem  VariantControl=OneThreePhaseBridge
  P : Outport  VectorParamsAs1DForOutWhenUnconnected=off

== system MMC_phase_hackathon_circuit4_HAAS_20260216/ /HB Twist M9/Twist Power Block/HRTimA_2/PWM Generator (2-Level)/Reference signal ==
  Uref : Inport
  External : Subsystem  VariantControl=External
  Internal : Subsystem  VariantControl=Internal
  Uref_In : Outport  VectorParamsAs1DForOutWhenUnconnected=off

== system MMC_phase_hackathon_circuit4_HAAS_20260216/ /HB Twist M9/Twist Power Block/HRTimA_2/PWM Generator (2-Level)/Sampling ==
  wt : Inport
  Uref : Inport  Port=2
  Sync Asymmetrical : Subsystem  VariantControl=SyncAsymmetrical
  Sync Natural : Subsystem  VariantControl=SyncNatural
  Sync Symmetrical : Subsystem  VariantControl=SyncSymmetrical
  Unsync Asymmetrical : Subsystem  VariantControl=UnsyncAsymmetrical
  Unsync Natural : Subsystem  VariantControl=UnsyncNatural
  Unsync Symmetrical : Subsystem  VariantControl=UnsyncSymmetrical
  Cr : Outport  VectorParamsAs1DForOutWhenUnconnected=off
  Uref* : Outport  Port=2  VectorParamsAs1DForOutWhenUnconnected=off

== system MMC_phase_hackathon_circuit4_HAAS_20260216/ /HB Twist M1/Twist Power Block/HRTimA_1/PWM Generator (2-Level)/Modulator type/Full Bridge Bipolar ==
  Cr : Inport
  Uref : Inport  Port=2
  Logical Operator : Logic  Operator=NOT  AllPortsSameDT=off  OutDataTypeStr=boolean
  Mux1 : Mux  Inputs=2
  Relational Operator2 : RelationalOperator  OutDataTypeStr=boolean
  Selector_FullBridgeIn : Selector  InputPortWidth=sps.SelectorFullBridgeIn_PortSize  IndexOptions=Index vector (dialog)  Indices=[1]  OutputSizes=1
  Selector_FullBridgeOut1 : Selector  InputPortWidth=2  IndexOptions=Index vector (dialog)  Indices=sps.SelectorFullBridgeOut_Index  OutputSizes=1
  P : Outport  SampleTime=Ts  VectorParamsAs1DForOutWhenUnconnected=off
  wires:
  Uref/1 -> Selector_FullBridgeIn/1
  Selector_FullBridgeIn/1 -> Relational Operator2/1
  Selector_FullBridgeOut1/1 -> P/1
  Cr/1 -> Relational Operator2/2
  Mux1/1 -> Selector_FullBridgeOut1/1
  Relational Operator2/1 -> Mux1/1, Logical Operator/1
  Logical Operator/1 -> Mux1/2

== system MMC_phase_hackathon_circuit4_HAAS_20260216/ /HB Twist M1/Twist Power Block/HRTimA_1/PWM Generator (2-Level)/Modulator type/Full Bridge Unipolar ==
  Cr : Inport
  Uref : Inport  Port=2
  Gain : Gain  Gain=-1
  Mux : Mux  Inputs=2
  Relational Operator1 : RelationalOperator  OutDataTypeStr=boolean
  Relational Operator3 : RelationalOperator  OutDataTypeStr=boolean
  Selector_FullBridgeIn : Selector  InputPortWidth=sps.SelectorFullBridgeIn_PortSize  IndexOptions=Index vector (dialog)  Indices=[1]  OutputSizes=1
  Selector_FullBridgeOut : Selector  InputPortWidth=2  IndexOptions=Index vector (dialog)  Indices=sps.SelectorFullBridgeOut_Index  OutputSizes=1
  P : Outport  SampleTime=Ts  VectorParamsAs1DForOutWhenUnconnected=off
  wires:
  Uref/1 -> Selector_FullBridgeIn/1
  Selector_FullBridgeIn/1 -> Relational Operator1/1, Gain/1
  Selector_FullBridgeOut/1 -> P/1
  Gain/1 -> Relational Operator3/1
  Relational Operator1/1 -> Mux/1
  Relational Operator3/1 -> Mux/2
  Mux/1 -> Selector_FullBridgeOut/1
  Cr/1 -> Relational Operator3/2, Relational Operator1/2

== system MMC_phase_hackathon_circuit4_HAAS_20260216/ /HB Twist M1/Twist Power Block/HRTimA_1/PWM Generator (2-Level)/Modulator type/One Three Phase Bridge ==
  Cr : Inport
  Uref : Inport  Port=2
  Relational Operator2 : RelationalOperator  OutDataTypeStr=boolean
  Selector_HalfBridgeOut : Selector  InputPortWidth=sps.SelectorHalfBridgeOut_PortSize  IndexOptions=Index vector (dialog)  Indices=sps.SelectorHalfBridgeOut_Index  OutputSizes=1
  P : Outport  PortDimensions=sps.SelectorHalfBridgeOut_PortSize  SampleTime=Ts  VectorParamsAs1DForOutWhenUnconnected=off
  wires:
  Uref/1 -> Relational Operator2/1
  Selector_HalfBridgeOut/1 -> P/1
  Cr/1 -> Relational Operator2/2
  Relational Operator2/1 -> Selector_HalfBridgeOut/1

== system MMC_phase_hackathon_circuit4_HAAS_20260216/ /HB Twist M1/Twist Power Block/HRTimA_1/PWM Generator (2-Level)/Reference signal/External ==
  Uref : Inport  PortDimensions=sps.UrefInport_PortDimensions  SampleTime=Ts
  Uref_In : Outport  VectorParamsAs1DForOutWhenUnconnected=off
  wires:
  Uref/1 -> Uref_In/1

== system MMC_phase_hackathon_circuit4_HAAS_20260216/ /HB Twist M1/Twist Power Block/HRTimA_1/PWM Generator (2-Level)/Reference signal/Internal ==
  Uref : Inport  PortDimensions=sps.UrefInport_PortDimensions  SampleTime=Ts
  Sine Wave : Sin  Amplitude=sps.m  Frequency=sps.Freq  Phase=sps.SinWave_Phase  SampleTime=Ts
  end : Terminator
  Uref_In : Outport  VectorParamsAs1DForOutWhenUnconnected=off
  wires:
  Sine Wave/1 -> Uref_In/1
  Uref/1 -> end/1

== system MMC_phase_hackathon_circuit4_HAAS_20260216/ /HB Twist M1/Twist Power Block/HRTimA_1/PWM Generator (2-Level)/Sampling/Sync Asymmetrical ==
  wt : Inport  Interpolate=off
  Uref : Inport  Port=2  Interpolate=off
  Add : Sum
  Add1 : Sum  Inputs=-+
  Constant3 : Constant
  Gain1 : Gain  Gain=2/pi  SaturateOnIntegerOverflow=on  OutDataTypeStr=Inherit: Same as input  ParamDataTypeStr=Inherit: Same as input
  Gain4 : Gain  Gain=nF  SaturateOnIntegerOverflow=on  OutDataTypeStr=Inherit: Same as input  ParamDataTypeStr=Inherit: Same as input
  Hit Crossing : HitCross  HitCrossingOffset=1e-9  HitCrossingDirection=falling
  Hit Crossing1 : HitCross  HitCrossingOffset=-1e-9  HitCrossingDirection=rising
  Logical Operator : Logic  Operator=OR  AllPortsSameDT=off  OutDataTypeStr=boolean
  Sample & Hold : Subsystem
  Trigonometric Function : Trigonometry  Operator=asin
  Trigonometric Function3 : Trigonometry
  Cr : Outport  VectorParamsAs1DForOutWhenUnconnected=off
  Uref* : Outport  Port=2  VectorParamsAs1DForOutWhenUnconnected=off
  wires:
  wt/1 -> Gain4/1
  Gain1/1 -> Cr/1, Add1/2, Add/1
  Trigonometric Function/1 -> Gain1/1
  Trigonometric Function3/1 -> Trigonometric Function/1
  Gain4/1 -> Trigonometric Function3/1
  Constant3/1 -> Add/2, Add1/1
  Add/1 -> Hit Crossing/1
  Add1/1 -> Hit Crossing1/1
  Uref/1 -> Sample & Hold/1(In)
  Sample & Hold/1(Out) -> Uref*/1
  Logical Operator/1 -> Sample & Hold/Enable
  Hit Crossing/1 -> Logical Operator/1
  Hit Crossing1/1 -> Logical Operator/2

== system MMC_phase_hackathon_circuit4_HAAS_20260216/ /HB Twist M1/Twist Power Block/HRTimA_1/PWM Generator (2-Level)/Sampling/Sync Natural ==
  wt : Inport
  Uref : Inport  Port=2
  Sync_NaturalSampling : Subsystem
  Cr : Outport  VectorParamsAs1DForOutWhenUnconnected=off
  Uref* : Outport  Port=2  VectorParamsAs1DForOutWhenUnconnected=off
  wires:
  Uref/1 -> Sync_NaturalSampling/1(Uref)
  wt/1 -> Sync_NaturalSampling/2(wt)
  Sync_NaturalSampling/1(Uref*) -> Uref*/1
  Sync_NaturalSampling/2(Cr) -> Cr/1

== system MMC_phase_hackathon_circuit4_HAAS_20260216/ /HB Twist M1/Twist Power Block/HRTimA_1/PWM Generator (2-Level)/Sampling/Sync Symmetrical ==
  wt : Inport
  Uref : Inport  Port=2
  Sync_SymmetricalSampling : Subsystem
  Cr : Outport  VectorParamsAs1DForOutWhenUnconnected=off
  Uref* : Outport  Port=2  VectorParamsAs1DForOutWhenUnconnected=off
  wires:
  Uref/1 -> Sync_SymmetricalSampling/1(Uref)
  wt/1 -> Sync_SymmetricalSampling/2(wt)
  Sync_SymmetricalSampling/1(Uref*) -> Uref*/1
  Sync_SymmetricalSampling/2(Cr) -> Cr/1

== system MMC_phase_hackathon_circuit4_HAAS_20260216/ /HB Twist M1/Twist Power Block/HRTimA_1/PWM Generator (2-Level)/Sampling/Unsync Asymmetrical ==
  wt : Inport
  Uref : Inport  Port=2
  Unsync_AsymmetricalSampling : Subsystem
  term1 : Terminator
  Cr : Outport  VectorParamsAs1DForOutWhenUnconnected=off
  Uref* : Outport  Port=2  VectorParamsAs1DForOutWhenUnconnected=off
  wires:
  Uref/1 -> Unsync_AsymmetricalSampling/1(Uref)
  Unsync_AsymmetricalSampling/1(Uref*) -> Uref*/1
  Unsync_AsymmetricalSampling/2(Cr) -> Cr/1
  wt/1 -> term1/1

== system MMC_phase_hackathon_circuit4_HAAS_20260216/ /HB Twist M1/Twist Power Block/HRTimA_1/PWM Generator (2-Level)/Sampling/Unsync Natural ==
  wt : Inport
  Uref : Inport  Port=2
  Unsync_NaturalSampling : Subsystem
  term1 : Terminator
  Cr : Outport  VectorParamsAs1DForOutWhenUnconnected=off
  Uref* : Outport  Port=2  VectorParamsAs1DForOutWhenUnconnected=off
  wires:
  Uref/1 -> Unsync_NaturalSampling/1(Uref)
  Unsync_NaturalSampling/1(Uref*) -> Uref*/1
  Unsync_NaturalSampling/2(Cr) -> Cr/1
  wt/1 -> term1/1

== system MMC_phase_hackathon_circuit4_HAAS_20260216/ /HB Twist M1/Twist Power Block/HRTimA_1/PWM Generator (2-Level)/Sampling/Unsync Symmetrical ==
  wt : Inport
  Uref : Inport  Port=2
  Unsync_SymmetricalSampling : Subsystem
  term1 : Terminator
  Cr : Outport  VectorParamsAs1DForOutWhenUnconnected=off
  Uref* : Outport  Port=2  VectorParamsAs1DForOutWhenUnconnected=off
  wires:
  Uref/1 -> Unsync_SymmetricalSampling/1(Uref)
  Unsync_SymmetricalSampling/1(Uref*) -> Uref*/1
  Unsync_SymmetricalSampling/2(Cr) -> Cr/1
  wt/1 -> term1/1

== system MMC_phase_hackathon_circuit4_HAAS_20260216/ /HB Twist M1/Twist Power Block/HRTimA_2/PWM Generator (2-Level)/Modulator type/Full Bridge Bipolar ==
  Cr : Inport
  Uref : Inport  Port=2
  Logical Operator : Logic  Operator=NOT  AllPortsSameDT=off  OutDataTypeStr=boolean
  Mux1 : Mux  Inputs=2
  Relational Operator2 : RelationalOperator  OutDataTypeStr=boolean
  Selector_FullBridgeIn : Selector  InputPortWidth=sps.SelectorFullBridgeIn_PortSize  IndexOptions=Index vector (dialog)  Indices=[1]  OutputSizes=1
  Selector_FullBridgeOut1 : Selector  InputPortWidth=2  IndexOptions=Index vector (dialog)  Indices=sps.SelectorFullBridgeOut_Index  OutputSizes=1
  P : Outport  SampleTime=Ts  VectorParamsAs1DForOutWhenUnconnected=off
  wires:
  Uref/1 -> Selector_FullBridgeIn/1
  Selector_FullBridgeIn/1 -> Relational Operator2/1
  Selector_FullBridgeOut1/1 -> P/1
  Cr/1 -> Relational Operator2/2
  Mux1/1 -> Selector_FullBridgeOut1/1
  Relational Operator2/1 -> Mux1/1, Logical Operator/1
  Logical Operator/1 -> Mux1/2

== system MMC_phase_hackathon_circuit4_HAAS_20260216/ /HB Twist M1/Twist Power Block/HRTimA_2/PWM Generator (2-Level)/Modulator type/Full Bridge Unipolar ==
  Cr : Inport
  Uref : Inport  Port=2
  Gain : Gain  Gain=-1
  Mux : Mux  Inputs=2
  Relational Operator1 : RelationalOperator  OutDataTypeStr=boolean
  Relational Operator3 : RelationalOperator  OutDataTypeStr=boolean
  Selector_FullBridgeIn : Selector  InputPortWidth=sps.SelectorFullBridgeIn_PortSize  IndexOptions=Index vector (dialog)  Indices=[1]  OutputSizes=1
  Selector_FullBridgeOut : Selector  InputPortWidth=2  IndexOptions=Index vector (dialog)  Indices=sps.SelectorFullBridgeOut_Index  OutputSizes=1
  P : Outport  SampleTime=Ts  VectorParamsAs1DForOutWhenUnconnected=off
  wires:
  Uref/1 -> Selector_FullBridgeIn/1
  Selector_FullBridgeIn/1 -> Relational Operator1/1, Gain/1
  Selector_FullBridgeOut/1 -> P/1
  Gain/1 -> Relational Operator3/1
  Relational Operator1/1 -> Mux/1
  Relational Operator3/1 -> Mux/2
  Mux/1 -> Selector_FullBridgeOut/1
  Cr/1 -> Relational Operator3/2, Relational Operator1/2

== system MMC_phase_hackathon_circuit4_HAAS_20260216/ /HB Twist M1/Twist Power Block/HRTimA_2/PWM Generator (2-Level)/Modulator type/One Three Phase Bridge ==
  Cr : Inport
  Uref : Inport  Port=2
  Relational Operator2 : RelationalOperator  OutDataTypeStr=boolean
  Selector_HalfBridgeOut : Selector  InputPortWidth=sps.SelectorHalfBridgeOut_PortSize  IndexOptions=Index vector (dialog)  Indices=sps.SelectorHalfBridgeOut_Index  OutputSizes=1
  P : Outport  PortDimensions=sps.SelectorHalfBridgeOut_PortSize  SampleTime=Ts  VectorParamsAs1DForOutWhenUnconnected=off
  wires:
  Uref/1 -> Relational Operator2/1
  Selector_HalfBridgeOut/1 -> P/1
  Cr/1 -> Relational Operator2/2
  Relational Operator2/1 -> Selector_HalfBridgeOut/1

== system MMC_phase_hackathon_circuit4_HAAS_20260216/ /HB Twist M1/Twist Power Block/HRTimA_2/PWM Generator (2-Level)/Reference signal/External ==
  Uref : Inport  PortDimensions=sps.UrefInport_PortDimensions  SampleTime=Ts
  Uref_In : Outport  VectorParamsAs1DForOutWhenUnconnected=off
  wires:
  Uref/1 -> Uref_In/1

== system MMC_phase_hackathon_circuit4_HAAS_20260216/ /HB Twist M1/Twist Power Block/HRTimA_2/PWM Generator (2-Level)/Reference signal/Internal ==
  Uref : Inport  PortDimensions=sps.UrefInport_PortDimensions  SampleTime=Ts
  Sine Wave : Sin  Amplitude=sps.m  Frequency=sps.Freq  Phase=sps.SinWave_Phase  SampleTime=Ts
  end : Terminator
  Uref_In : Outport  VectorParamsAs1DForOutWhenUnconnected=off
  wires:
  Sine Wave/1 -> Uref_In/1
  Uref/1 -> end/1
